simulink subsystem "TV_FLC_V2"  (R2026a)
settings: Solver=VariableStepAuto
model mask{MotorT=Control.MotorTrq, Gr=Control.GearRatio, MotorW=Control.MotorW, rwheel=Control.WheelRad, tr=Control.RearTrack, a=Control.FrontTrackToCG, a_cop=Control.FrontTrackToCoP, Af=Control.FrontalArea, cd=Control.LiftCoef, g=Control.GravitationalAcc, ro=Control.AirDensity, m=Control.Mass, h_CG=Control.CGHeight, L=Control.Wheelbase, Gain=aSteerRatio, Ku=Control.Ku, F=Control.F, P=Control.Proportional_P, I=Control.Integral_I, D=Control.Derivative_D, N=0, Load_Ref=Control.LoadRef, Slip_Ref=Control.SlipRef, FIS_1=Control.FuzzySystem, FIS_2=0, FIS_3=0, vx_th=vx_th, Tmax=max(Control.MotorTrq), C_alpha_F=Control.CalphaF}
  mask prompts: MotorT "Motor Torque:"; Gr "Gear Ratio:"; MotorW "Motor RPM:"; rwheel "Wheel Radius:"; tr "Rear Track:"; a "Front Track to CG:"; a_cop "Front Track to CoP"; Af "Frontal Area:"; cd "Lift Coef:"; g "Graviational ACc"; ro "Air Density:"; m "Mass:"; h_CG "CG Height:"; L "Wheelbase:"; Gain "Simulink:blkprm_prompts:GainGain"; Ku "Understeer Gradient:"; F "Moment to Torque"; P "Simulink:masks:ProportionalP_MP"; I "Simulink:masks:IntegralI_MP"; D "Simulink:masks:DerivativeD_MP"; N "Filter (N):"; Load_Ref "Reference Load Table:"; Slip_Ref "Reference Slip Table:"; FIS_1 "Fuzzy Inference System Var1:"; FIS_2 "Fuzzy Inference System Var2:"; FIS_3 "Fuzzy Inference System Var3:"; vx_th "Activation Velocity:"; Tmax "Max Torque"; C_alpha_F "Front Cornering Stiffness:"
values from neighbouring files (symbols this model uses):
  a = -Vehicle.Chassis.Body.sCG.Value(1)    [sm_car_controlparam_FLCDYC_V2.m]
  Gr = 1/Vehicle.Powertrain.Driveline.Gearbox.ratio.Value    [sm_car_controlparam_FLCDYC_V2.m]
  L = 1.578    [sm_car_controlparam_FLCDYC_V2.m]
  rwheel = 0.263    [sm_car_controlparam_FLCDYC_V2.m]
  tr = Vehicle.Chassis.Body.TrackRear.Value    [sm_car_controlparam_FLCDYC_V2.m]
libraries: simulink x4, fuzblock x3, slpidlib x2, sl_discontinuities x1
settings Model: Creator=andrei  LastModifiedBy=andrei

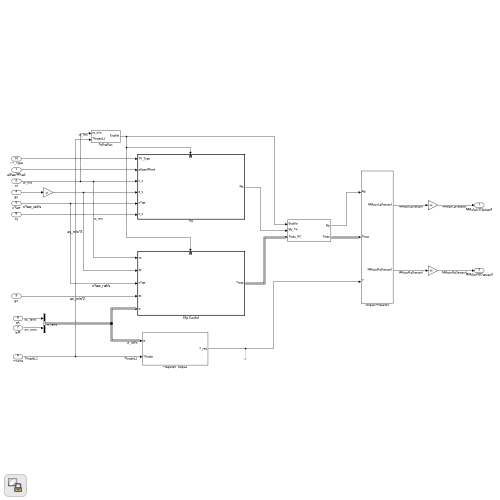
[thumbnail: Simulink's stored preview of the top-level diagram]
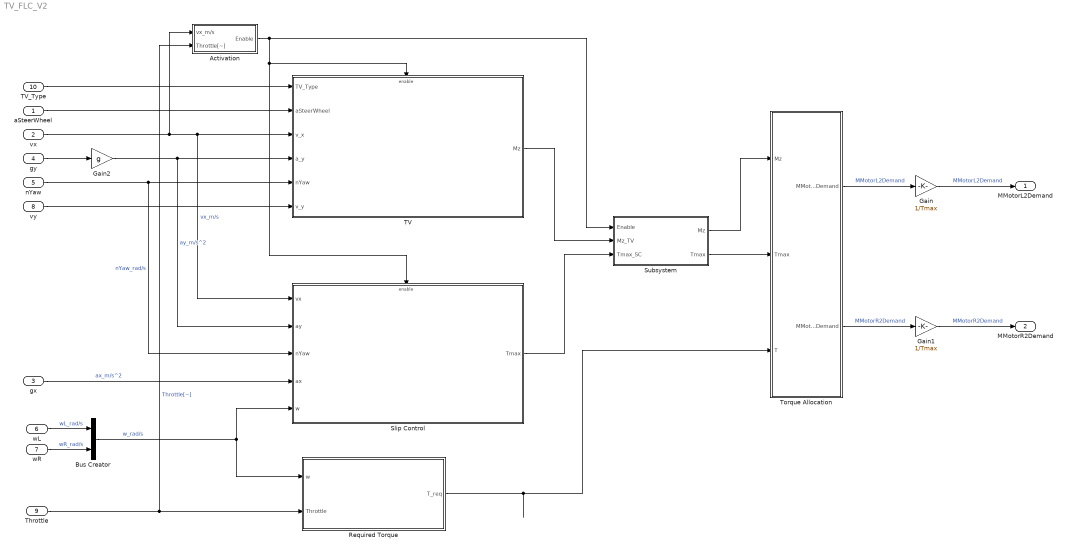
== system TV_FLC_V2 ==
  aSteerWheel : Inport  OutDataTypeStr=double  PortDimensions=1  SampleTime=0
  vx : Inport  Port=2  OutDataTypeStr=double  PortDimensions=1  SampleTime=0
  gx : Inport  Port=3  OutDataTypeStr=double  PortDimensions=1  SampleTime=0
  gy : Inport  Port=4  OutDataTypeStr=double  PortDimensions=1  SampleTime=0
  nYaw : Inport  Port=5  OutDataTypeStr=double  PortDimensions=1  SampleTime=0
  wL : Inport  Port=6  OutDataTypeStr=double  PortDimensions=1  SampleTime=0
  wR : Inport  Port=7  OutDataTypeStr=double  PortDimensions=1  SampleTime=0
  vy : Inport  Port=8  OutDataTypeStr=double  PortDimensions=1  SampleTime=0
  Throttle : Inport  Port=9  OutDataTypeStr=double  PortDimensions=1  SampleTime=0
  TV_Type : Inport  Port=10  OutDataTypeStr=double  PortDimensions=1  SampleTime=0
  Activation : Subsystem
  Bus Creator : BusCreator  Inputs=2
  Gain : Gain  Gain=1/Tmax
  Gain1 : Gain  Gain=1/Tmax
  Gain2 : Gain  Gain=g
  Required Torque : Subsystem
  Slip Control : Subsystem
  Subsystem : Subsystem
  TV : Subsystem
  Torque Allocation : Subsystem
  MMotorL2Demand : Outport  OutDataTypeStr=double  PortDimensions=1  SampleTime=0
  MMotorR2Demand : Outport  Port=2  OutDataTypeStr=double  PortDimensions=1  SampleTime=0
  wires:
  Torque Allocation/1(MMotorL2Demand) -> Gain/1  "MMotorL2Demand"
  wL/1 -> Bus Creator/1  "wL_rad/s"
  gy/1 -> Gain2/1
  Gain1/1 -> MMotorR2Demand/1  "MMotorR2Demand"
  Gain/1 -> MMotorL2Demand/1  "MMotorL2Demand"
  Torque Allocation/2(MMotorR2Demand) -> Gain1/1  "MMotorR2Demand"
  wR/1 -> Bus Creator/2  "wR_rad/s"
  Slip Control/1(Tmax) -> Subsystem/3(Tmax_SC)
  Required Torque/1(T_req) -> Torque Allocation/3(T)
  aSteerWheel/1 -> TV/2(aSteerWheel)
  Gain2/1 -> TV/4(a_y), Slip Control/2(ay)  "ay_m/s^2"
  Bus Creator/1 -> Slip Control/5(w), Required Torque/1(w)  "w_rad/s"
  nYaw/1 -> TV/5(nYaw), Slip Control/3(nYaw)  "nYaw_rad/s"
  gx/1 -> Slip Control/4(ax)  "ax_m/s^2"
  Throttle/1 -> Activation/2(Throttle[~]), Required Torque/2(Throttle)  "Throttle[~]"
  TV/1(Mz) -> Subsystem/2(Mz_TV)
  vy/1 -> TV/6(v_y)
  vx/1 -> TV/3(v_x), Slip Control/1(vx), Activation/1(vx_m/s)  "vx_m/s"
  Activation/1(Enable) -> Slip Control/Enable, TV/Enable, Subsystem/1(Enable)
  Subsystem/1(Mz) -> Torque Allocation/1(Mz)
  Subsystem/2(Tmax) -> Torque Allocation/2(Tmax)
  TV_Type/1 -> TV/1(TV_Type)

== system TV_FLC_V2/Activation ==
  vx_m/s : Inport
  Throttle[~] : Inport  Port=2
  AND : Logic  AllPortsSameDT=off  OutDataTypeStr=boolean
  Compare To Zero : simulink/Logic and Bit Operations/Compare To Zero  relop=~=  OutDataTypeStr=boolean
  Relational Operator : RelationalOperator  Operator=<=  OutDataTypeStr=boolean  RndMeth=Simplest  InputSameDT=off
  th_vx_min : Constant  Value=vx_th
  Enable : Outport
  wires:
  Compare To Zero/1 -> AND/2
  AND/1 -> Enable/1
  Throttle[~]/1 -> Compare To Zero/1
  th_vx_min/1 -> Relational Operator/1
  vx_m/s/1 -> Relational Operator/2
  Relational Operator/1 -> AND/1

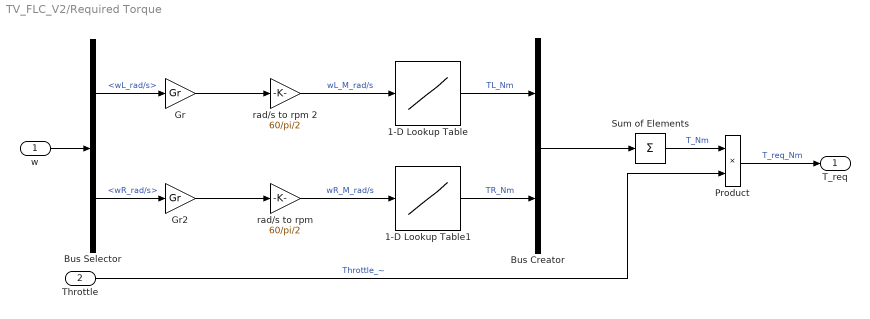
== system TV_FLC_V2/Required Torque ==
  w : Inport
  Throttle : Inport  Port=2
  1-D Lookup Table : Lookup_n-D  NumberOfTableDimensions=1  BreakpointsForDimension1=MotorW  Table=MotorT  InternalRulePriority=Speed  RndMeth=Simplest
  1-D Lookup Table1 : Lookup_n-D  NumberOfTableDimensions=1  BreakpointsForDimension1=MotorW  Table=MotorT  InternalRulePriority=Speed  RndMeth=Simplest
  Bus Creator : BusCreator  Inputs=2
  Bus Selector : BusSelector  OutputSignals=wL_rad/s,wR_rad/s
  Gr : Gain  Gain=Gr
  Gr2 : Gain  Gain=Gr
  Product : Product
  Sum of Elements : Sum  Inputs=+
  rad/s to rpm : Gain  Gain=60/pi/2
  rad/s to rpm 2 : Gain  Gain=60/pi/2
  T_req : Outport
  wires:
  Gr2/1 -> rad/s to rpm/1
  Gr/1 -> rad/s to rpm 2/1
  Bus Creator/1 -> Sum of Elements/1
  1-D Lookup Table/1 -> Bus Creator/1  "TL_Nm"
  rad/s to rpm 2/1 -> 1-D Lookup Table/1  "wL_M_rad/s"
  Bus Selector/2 -> Gr2/1  "<wR_rad/s>"
  Product/1 -> T_req/1  "T_req_Nm"
  Bus Selector/1 -> Gr/1  "<wL_rad/s>"
  rad/s to rpm/1 -> 1-D Lookup Table1/1  "wR_M_rad/s"
  Throttle/1 -> Product/2  "Throttle_~"
  1-D Lookup Table1/1 -> Bus Creator/2  "TR_Nm"
  Sum of Elements/1 -> Product/1  "T_Nm"
  w/1 -> Bus Selector/1

== system TV_FLC_V2/Slip Control ==
  vx : Inport
  ay : Inport  Port=2
  nYaw : Inport  Port=3
  ax : Inport  Port=4
  w : Inport  Port=5
  Enable : EnablePort  StatesWhenEnabling=reset
  Loads : Subsystem
  Maximum Torque Allowed : Subsystem
  Slip Calculation : Subsystem
  Tmax : Outport
  wires:
  w/1 -> Slip Calculation/3(w)  "w_rad/s"
  nYaw/1 -> Slip Calculation/2(nYaw)  "nYaw_rad/s"
  ax/1 -> Loads/1(ax)  "ax_m/s^2"
  Loads/1(Fz) -> Maximum Torque Allowed/1(Fz)
  ay/1 -> Loads/2(ay)  "ay_m/s^2"
  Slip Calculation/2(kappa_rr) -> Maximum Torque Allowed/3(kappa_rr)
  vx/1 -> Loads/3(vx), Slip Calculation/1(Vx)  "vx_m/s"
  Maximum Torque Allowed/1(Tmax) -> Tmax/1
  Slip Calculation/1(kappa_rl) -> Maximum Torque Allowed/2(kappa_rl)

== system TV_FLC_V2/Subsystem ==
  Enable : Inport
  Mz_TV : Inport  Port=2
  Tmax_SC : Inport  Port=3
  Bus Creator1 : BusCreator  Inputs=2
  Constant : Constant  Value=Tmax
  Constant1 : Constant  Value=Tmax
  Constant2 : Constant  Value=0
  Switch : Switch  Criteria=u2 ~= 0  SaturateOnIntegerOverflow=off  InputSameDT=off
  Switch1 : Switch  Criteria=u2 ~= 0  SaturateOnIntegerOverflow=off  InputSameDT=off
  Mz : Outport
  Tmax : Outport  Port=2
  wires:
  Switch1/1 -> Mz/1
  Constant2/1 -> Switch1/3  "Mz"
  Mz_TV/1 -> Switch1/1
  Constant/1 -> Bus Creator1/1  "Tmax_rl_Nm"
  Tmax_SC/1 -> Switch/1
  Bus Creator1/1 -> Switch/3
  Switch/1 -> Tmax/1
  Constant1/1 -> Bus Creator1/2  "Tmax_rr_Nm"
  Enable/1 -> Switch/2, Switch1/2

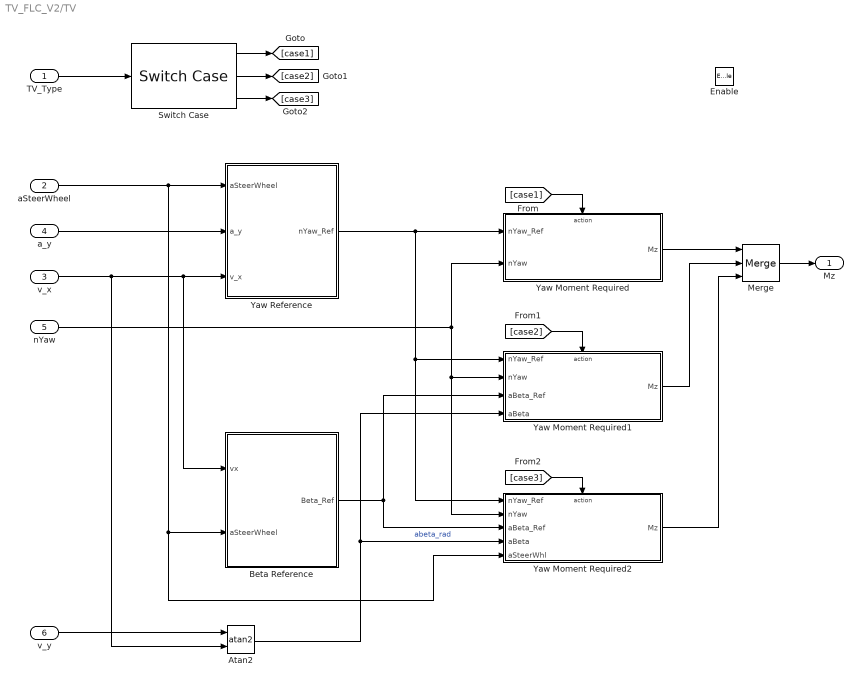
== system TV_FLC_V2/TV ==
  TV_Type : Inport
  aSteerWheel : Inport  Port=2
  v_x : Inport  Port=3
  a_y : Inport  Port=4
  nYaw : Inport  Port=5
  v_y : Inport  Port=6
  Enable : EnablePort  StatesWhenEnabling=reset
  Atan2 : Trigonometry  Operator=atan2
  Beta Reference : Subsystem
  Merge : Merge  Inputs=3
  Switch Case : SwitchCase  CaseConditions={1, 2, 3}  ShowDefaultCase=off
  Yaw Moment Required : Subsystem
  Yaw Moment Required1 : Subsystem
  Yaw Moment Required2 : Subsystem
  Yaw Reference : Subsystem
  Mz : Outport
  wires:
  [case2] -> Yaw Moment Required1/Action
  Merge/1 -> Mz/1
  Yaw Moment Required2/1(Mz) -> Merge/3
  [case3] -> Yaw Moment Required2/Action
  Switch Case/3 -> [case3]
  Switch Case/2 -> [case2]
  [case1] -> Yaw Moment Required/Action
  Switch Case/1 -> [case1]
  Atan2/1 -> Yaw Moment Required2/4(aBeta), Yaw Moment Required1/4(aBeta)  "abeta_rad"
  Yaw Moment Required1/1(Mz) -> Merge/2
  TV_Type/1 -> Switch Case/1
  aSteerWheel/1 -> Yaw Moment Required2/5(aSteerWhl), Beta Reference/2(aSteerWheel), Yaw Reference/1(aSteerWheel)
  v_x/1 -> Yaw Reference/3(v_x), Beta Reference/1(vx), Atan2/2
  nYaw/1 -> Yaw Moment Required1/2(nYaw), Yaw Moment Required2/2(nYaw), Yaw Moment Required/2(nYaw)
  a_y/1 -> Yaw Reference/2(a_y)
  Yaw Moment Required/1(Mz) -> Merge/1
  Yaw Reference/1(nYaw_Ref) -> Yaw Moment Required1/1(nYaw_Ref), Yaw Moment Required2/1(nYaw_Ref), Yaw Moment Required/1(nYaw_Ref)
  Beta Reference/1(Beta_Ref) -> Yaw Moment Required2/3(aBeta_Ref), Yaw Moment Required1/3(aBeta_Ref)
  v_y/1 -> Atan2/1

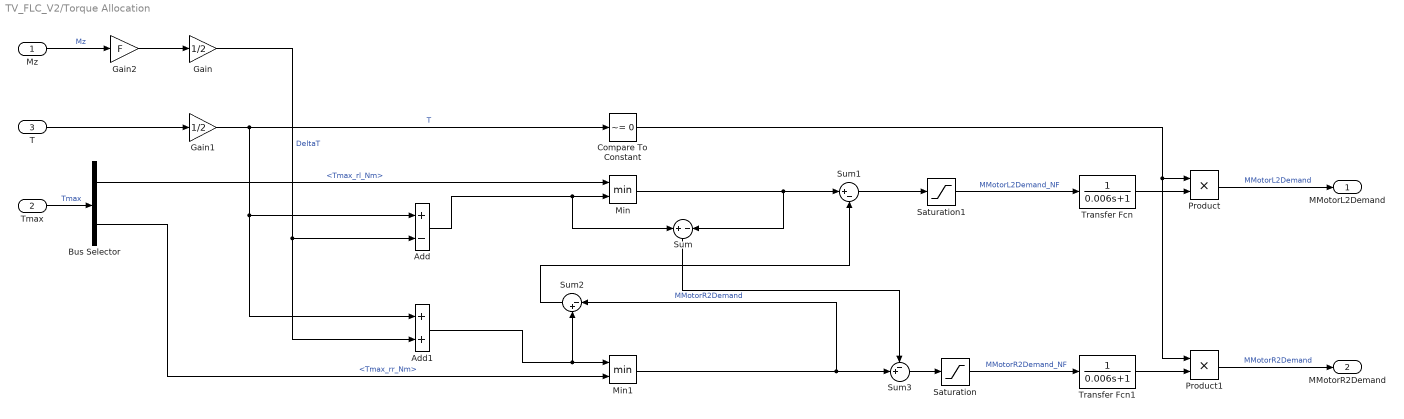
== system TV_FLC_V2/Torque Allocation ==
  Mz : Inport
  Tmax : Inport  Port=2
  T : Inport  Port=3
  Add : Sum  Inputs=+-
  Add1 : Sum
  Bus Selector : BusSelector  OutputSignals=Tmax_rl_Nm,Tmax_rr_Nm
  Compare To Constant : simulink/Logic and Bit Operations/Compare To Constant  relop=~=  const=0  OutDataTypeStr=boolean
  Gain : Gain  Gain=1/2
  Gain1 : Gain  Gain=1/2
  Gain2 : Gain  Gain=F
  Min : MinMax  Inputs=2
  Min1 : MinMax  Inputs=2
  Product : Product
  Product1 : Product
  Saturation : Saturate  UpperLimit=Tmax  LowerLimit=0
  Saturation1 : Saturate  UpperLimit=Tmax  LowerLimit=0
  Sum : Sum  Inputs=+|-
  Sum1 : Sum  Inputs=|+-
  Sum2 : Sum  Inputs=|-+
  Sum3 : Sum  Inputs=-+|
  Transfer Fcn : TransferFcn  Denominator=[0.006 1]
  Transfer Fcn1 : TransferFcn  Denominator=[0.006 1]
  MMotorL2Demand : Outport
  MMotorR2Demand : Outport  Port=2
  wires:
  Saturation1/1 -> Transfer Fcn/1  "MMotorL2Demand_NF"
  Sum3/1 -> Saturation/1
  Sum1/1 -> Saturation1/1
  Gain2/1 -> Gain/1
  Gain/1 -> Add1/2, Add/2  "DeltaT"
  T/1 -> Gain1/1
  Mz/1 -> Gain2/1  "Mz"
  Min/1 -> Sum1/1, Sum/2
  Min1/1 -> Sum2/1, Sum3/2  "MMotorR2Demand"
  Tmax/1 -> Bus Selector/1  "Tmax"
  Bus Selector/1 -> Min/1  "<Tmax_rl_Nm>"
  Bus Selector/2 -> Min1/2  "<Tmax_rr_Nm>"
  Add/1 -> Sum/1, Min/2
  Add1/1 -> Sum2/2, Min1/1
  Sum2/1 -> Sum1/2
  Sum/1 -> Sum3/1
  Gain1/1 -> Compare To Constant/1, Add1/1, Add/1  "T"
  Compare To Constant/1 -> Product/1, Product1/1
  Transfer Fcn/1 -> Product/2
  Product/1 -> MMotorL2Demand/1  "MMotorL2Demand"
  Saturation/1 -> Transfer Fcn1/1  "MMotorR2Demand_NF"
  Transfer Fcn1/1 -> Product1/2
  Product1/1 -> MMotorR2Demand/1  "MMotorR2Demand"

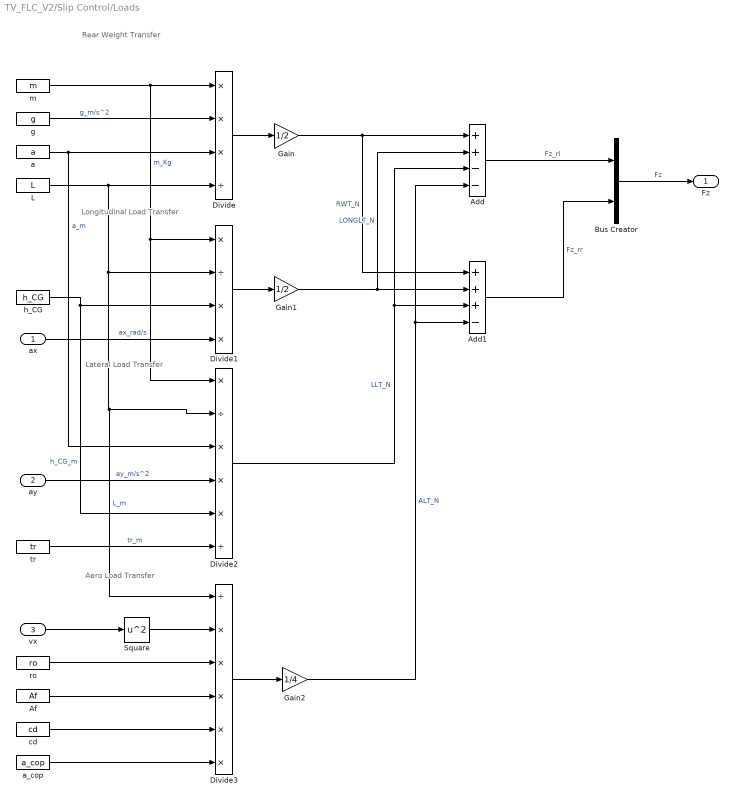
== system TV_FLC_V2/Slip Control/Loads ==
  note: Aero Load Transfer
  note: Lateral Load Transfer
  note: Longitudinal Load Transfer
  note: Rear Weight Transfer
  ax : Inport
  ay : Inport  Port=2
  vx : Inport  Port=3
  Add : Sum  Inputs=++--
  Add1 : Sum  Inputs=+++-
  Af : Constant  Value=Af
  Bus Creator : BusCreator  Inputs=2
  Divide : Product  Inputs=***/
  Divide1 : Product  Inputs=*/**
  Divide2 : Product  Inputs=*/***/
  Divide3 : Product  Inputs=/*****
  Gain : Gain  Gain=1/2
  Gain1 : Gain  Gain=1/2
  Gain2 : Gain  Gain=1/4
  L : Constant  Value=L
  Square : Math  Operator=square
  a : Constant  Value=a
  a_cop : Constant  Value=a_cop
  cd : Constant  Value=cd
  g : Constant  Value=g
  h_CG : Constant  Value=h_CG
  m : Constant  Value=m
  ro : Constant  Value=ro
  tr : Constant  Value=tr
  Fz : Outport
  wires:
  m/1 -> Divide/1, Divide1/1, Divide2/1  "m_Kg"
  g/1 -> Divide/2  "g_m/s^2"
  a/1 -> Divide/3, Divide2/3  "a_m"
  L/1 -> Divide3/1, Divide2/2, Divide1/2, Divide/4  "L_m"
  Divide/1 -> Gain/1
  vx/1 -> Square/1
  Square/1 -> Divide3/2
  Gain/1 -> Add/1, Add1/1  "RWT_N"
  Gain2/1 -> Add/4, Add1/4  "ALT_N"
  h_CG/1 -> Divide2/5, Divide1/3  "h_CG_m"
  ax/1 -> Divide1/4  "ax_rad/s"
  Divide1/1 -> Gain1/1
  Gain1/1 -> Add/2, Add1/2  "LONGLT_N"
  ay/1 -> Divide2/4  "ay_m/s^2"
  tr/1 -> Divide2/6  "tr_m"
  Divide2/1 -> Add/3, Add1/3  "LLT_N"
  Add/1 -> Bus Creator/1  "Fz_rl"
  Add1/1 -> Bus Creator/2  "Fz_rr"
  Bus Creator/1 -> Fz/1  "Fz"
  Divide3/1 -> Gain2/1
  ro/1 -> Divide3/3
  Af/1 -> Divide3/4
  cd/1 -> Divide3/5
  a_cop/1 -> Divide3/6

== system TV_FLC_V2/Slip Control/Maximum Torque Allowed ==
  Fz : Inport
  kappa_rl : Inport  Port=2
  kappa_rr : Inport  Port=3
  Bus Creator : BusCreator  Inputs=2
  Bus Selector : BusSelector  OutputSignals=Fz_rl,Fz_rr
  Slip Correction Left : Subsystem
  Slip Correction Right : Subsystem
  Tmax : Outport
  wires:
  Slip Correction Right/1(Tmax_rr) -> Bus Creator/2  "Tmax_rr_Nm"
  Slip Correction Left/1(Tmax_rl) -> Bus Creator/1  "Tmax_rl_Nm"
  kappa_rl/1 -> Slip Correction Left/1(kappa_rl)
  kappa_rr/1 -> Slip Correction Right/2(kappa_rr)
  Fz/1 -> Bus Selector/1
  Bus Selector/1 -> Slip Correction Left/2(Fz_rl)  "<Fz_rl>"
  Bus Selector/2 -> Slip Correction Right/1(Fz_rr)  "<Fz_rr>"
  Bus Creator/1 -> Tmax/1

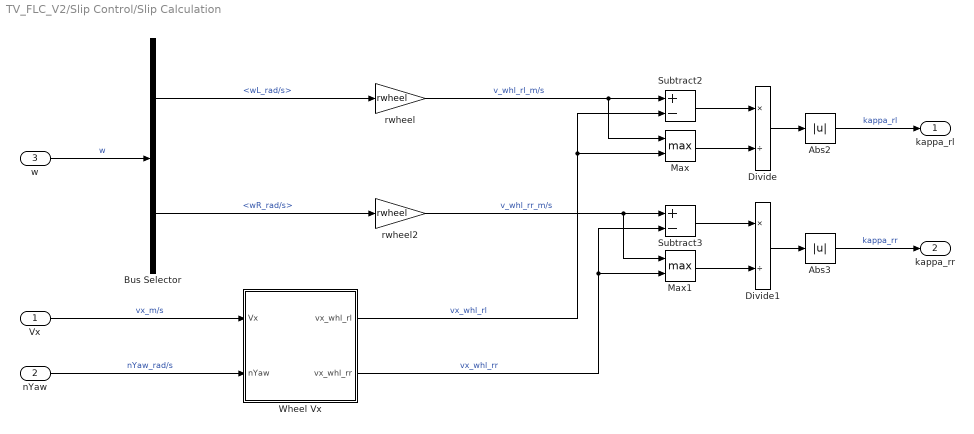
== system TV_FLC_V2/Slip Control/Slip Calculation ==
  Vx : Inport
  nYaw : Inport  Port=2
  w : Inport  Port=3
  Abs2 : Abs  SaturateOnIntegerOverflow=off
  Abs3 : Abs  SaturateOnIntegerOverflow=off
  Bus Selector : BusSelector  OutputSignals=wL_rad/s,wR_rad/s
  Divide : Product  Inputs=*/
  Divide1 : Product  Inputs=*/
  Max : MinMax  Function=max  Inputs=2
  Max1 : MinMax  Function=max  Inputs=2
  Subtract2 : Sum  Inputs=+-
  Subtract3 : Sum  Inputs=+-
  Wheel Vx : Subsystem
  rwheel : Gain  Gain=rwheel
  rwheel2 : Gain  Gain=rwheel
  kappa_rl : Outport
  kappa_rr : Outport  Port=2
  wires:
  Bus Selector/1 -> rwheel/1  "<wL_rad/s>"
  Bus Selector/2 -> rwheel2/1  "<wR_rad/s>"
  Vx/1 -> Wheel Vx/1(Vx)  "vx_m/s"
  w/1 -> Bus Selector/1  "w"
  rwheel/1 -> Max/1, Subtract2/1  "v_whl_rl_m/s"
  rwheel2/1 -> Max1/1, Subtract3/1  "v_whl_rr_m/s"
  nYaw/1 -> Wheel Vx/2(nYaw)  "nYaw_rad/s"
  Abs3/1 -> kappa_rr/1  "kappa_rr"
  Wheel Vx/1(vx_whl_rl) -> Subtract2/2, Max/2  "vx_whl_rl"
  Abs2/1 -> kappa_rl/1  "kappa_rl"
  Subtract2/1 -> Divide/1
  Wheel Vx/2(vx_whl_rr) -> Subtract3/2, Max1/2  "vx_whl_rr"
  Subtract3/1 -> Divide1/1
  Divide/1 -> Abs2/1
  Max/1 -> Divide/2
  Divide1/1 -> Abs3/1
  Max1/1 -> Divide1/2

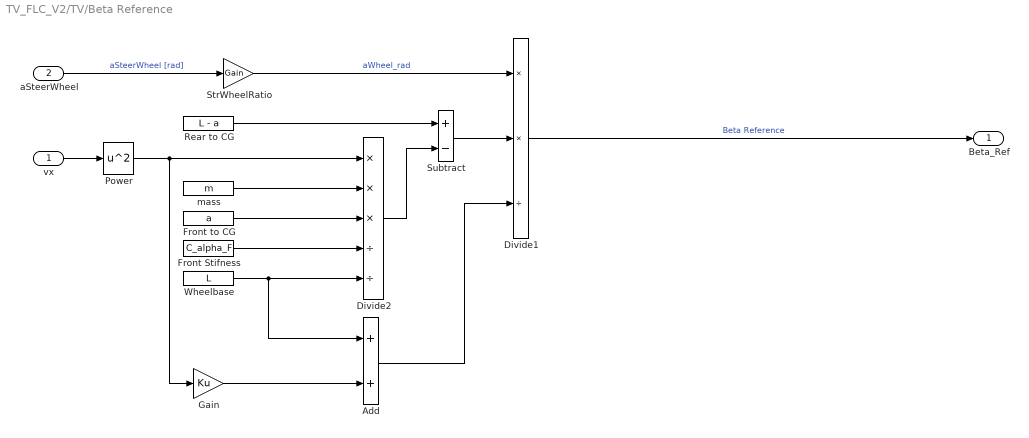
== system TV_FLC_V2/TV/Beta Reference ==
  vx : Inport
  aSteerWheel : Inport  Port=2
  Add : Sum
  Divide1 : Product  Inputs=**/
  Divide2 : Product  Inputs=***//
  Front Stifness : Constant  Value=C_alpha_F
  Front to CG : Constant  Value=a
  Gain : Gain  Gain=Ku
  Power : Math  Operator=square
  Rear to CG : Constant  Value=L - a
  StrWheelRatio : Gain  Gain=Gain
  Subtract : Sum  Inputs=+-
  Wheelbase : Constant  Value=L
  mass : Constant  Value=m
  Beta_Ref : Outport
  wires:
  StrWheelRatio/1 -> Divide1/1  "aWheel_rad"
  Add/1 -> Divide1/3
  Gain/1 -> Add/2
  Power/1 -> Gain/1, Divide2/1
  Divide1/1 -> Beta_Ref/1  "Beta Reference"
  vx/1 -> Power/1
  aSteerWheel/1 -> StrWheelRatio/1  "aSteerWheel [rad]"
  Wheelbase/1 -> Add/1, Divide2/5
  Front Stifness/1 -> Divide2/4
  mass/1 -> Divide2/2
  Front to CG/1 -> Divide2/3
  Rear to CG/1 -> Subtract/1
  Divide2/1 -> Subtract/2
  Subtract/1 -> Divide1/2

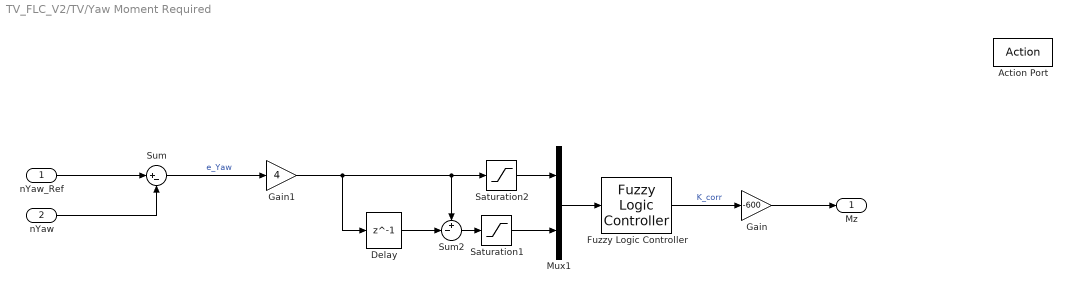
== system TV_FLC_V2/TV/Yaw Moment Required ==
  nYaw_Ref : Inport
  nYaw : Inport  Port=2
  Action Port : ActionPort
  Delay : Delay  DelayLength=1  InputProcessing=Columns as channels (frame based)
  Fuzzy Logic Controller : fuzblock/Fuzzy Logic  Controller  FIS=FIS_1  OutputSampleNumber=101  DataType=double  UseLookupTable=off  NumBreakpoints=10  FuzzifiedInputs=off  RuleFiringStrengths=off  RuleOutputs=off  AggregatedOutputs=off  SimulateUsing=Interpreted execution  OutOfRangeInputValueMessage=warning  NoRuleFiredMessage=warning  EmptyOutputFuzzySetMessage=warning
  Gain : Gain  Gain=-600
  Gain1 : Gain  Gain=4
  Mux1 : Mux  Inputs=2
  Saturation1 : Saturate  UpperLimit=1  LowerLimit=-1  ZeroCross=off
  Saturation2 : Saturate  UpperLimit=1  LowerLimit=-1  ZeroCross=off
  Sum : Sum  Inputs=|+-
  Sum2 : Sum  Inputs=+-|
  Mz : Outport
  wires:
  Gain1/1 -> Delay/1, Saturation2/1, Sum2/1
  Mux1/1 -> Fuzzy Logic Controller/1
  Sum2/1 -> Saturation1/1
  Delay/1 -> Sum2/2
  Saturation2/1 -> Mux1/1
  Saturation1/1 -> Mux1/2
  Gain/1 -> Mz/1
  Fuzzy Logic Controller/1 -> Gain/1  "K_corr"
  nYaw_Ref/1 -> Sum/1
  nYaw/1 -> Sum/2
  Sum/1 -> Gain1/1  "e_Yaw"

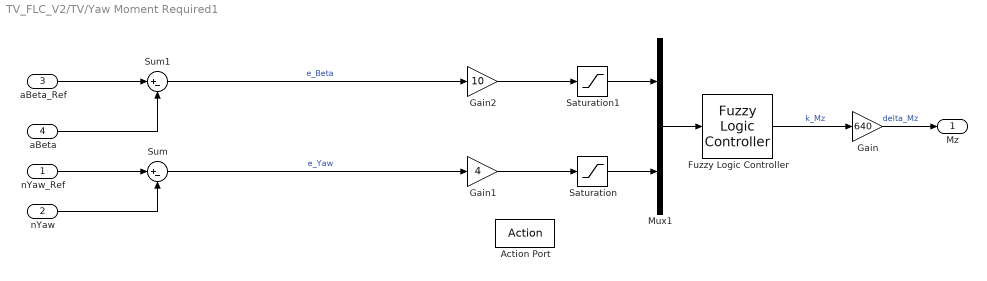
== system TV_FLC_V2/TV/Yaw Moment Required1 ==
  nYaw_Ref : Inport
  nYaw : Inport  Port=2
  aBeta_Ref : Inport  Port=3
  aBeta : Inport  Port=4
  Action Port : ActionPort
  Fuzzy Logic Controller : fuzblock/Fuzzy Logic  Controller  FIS=FIS_2  OutputSampleNumber=101  DataType=double  UseLookupTable=off  NumBreakpoints=10  FuzzifiedInputs=off  RuleFiringStrengths=off  RuleOutputs=off  AggregatedOutputs=off  SimulateUsing=Interpreted execution  OutOfRangeInputValueMessage=warning  NoRuleFiredMessage=warning  EmptyOutputFuzzySetMessage=warning
  Gain : Gain  Gain=640
  Gain1 : Gain  Gain=4
  Gain2 : Gain  Gain=10
  Mux1 : Mux  Inputs=2
  Saturation : Saturate  UpperLimit=1  LowerLimit=-1  ZeroCross=off
  Saturation1 : Saturate  UpperLimit=1  LowerLimit=-1  ZeroCross=off
  Sum : Sum  Inputs=|+-
  Sum1 : Sum  Inputs=|+-
  Mz : Outport
  wires:
  Saturation1/1 -> Mux1/1
  Saturation/1 -> Mux1/2
  Sum1/1 -> Gain2/1  "e_Beta"
  aBeta/1 -> Sum1/2
  aBeta_Ref/1 -> Sum1/1
  Sum/1 -> Gain1/1  "e_Yaw"
  nYaw/1 -> Sum/2
  nYaw_Ref/1 -> Sum/1
  Fuzzy Logic Controller/1 -> Gain/1  "k_Mz"
  Gain/1 -> Mz/1  "delta_Mz"
  Mux1/1 -> Fuzzy Logic Controller/1
  Gain2/1 -> Saturation1/1
  Gain1/1 -> Saturation/1

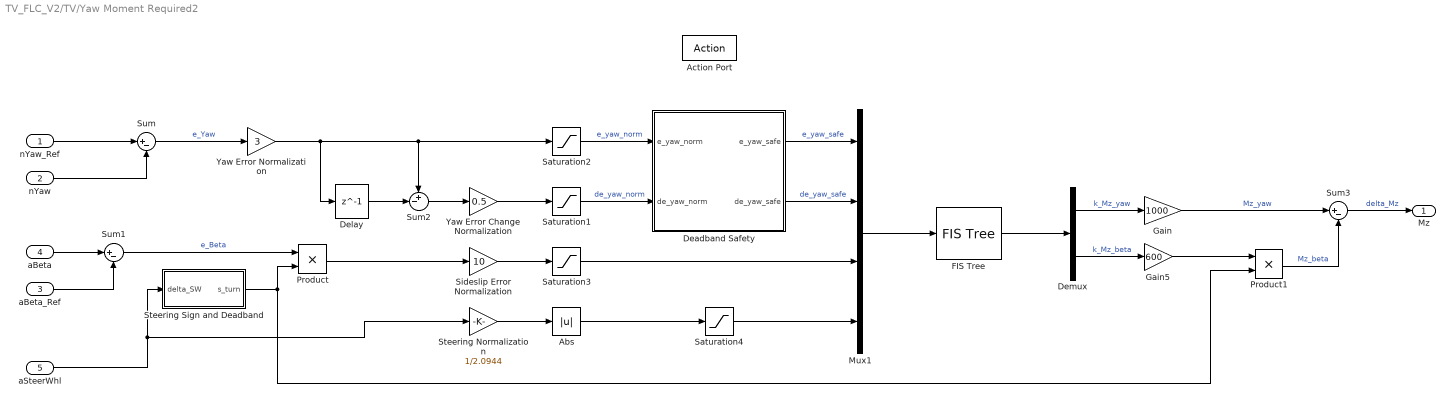
== system TV_FLC_V2/TV/Yaw Moment Required2 ==
  nYaw_Ref : Inport
  nYaw : Inport  Port=2
  aBeta_Ref : Inport  Port=3
  aBeta : Inport  Port=4
  aSteerWhl : Inport  Port=5
  Action Port : ActionPort
  " Yaw Error Change Normalization" : Gain  Gain=0.5
  Abs : Abs  ZeroCross=off  SaturateOnIntegerOverflow=off
  Deadband Safety : Subsystem
  Delay : Delay  DelayLength=1  InputProcessing=Columns as channels (frame based)
  Demux : Demux  Outputs=2
  FIS Tree : fuzblock/FIS Tree  FIS=FIS_3  OutputSampleNumber=101  DataType=single  SimulateUsing=Interpreted execution  OutOfRangeInputValueMessage=warning  NoRuleFiredMessage=warning  EmptyOutputFuzzySetMessage=warning
  Gain : Gain  Gain=1000
  Gain5 : Gain  Gain=600
  Mux1 : Mux
  Product : Product
  Product1 : Product
  Saturation{1..4} (4 alike) : Saturate  UpperLimit=1  LowerLimit=-1  ZeroCross=off
  Sideslip Error Normalization : Gain  Gain=10
  Steering Normalization : Gain  Gain=1/2.0944
  Steering Sign and Deadband : MATLAB Function  TreatAsAtomicUnit=on  mask{delta_th=2}
      mask prompts: delta_th "Steering Th"
  Sum : Sum  Inputs=|+-
  Sum1 : Sum  Inputs=|+-
  Sum2 : Sum  Inputs=+-|
  Sum3 : Sum  Inputs=|+-
  Yaw Error Normalization : Gain  Gain=3
  Mz : Outport
  wires:
  Deadband Safety/2(de_yaw_safe) -> Mux1/2  "de_yaw_safe"
  Deadband Safety/1(e_yaw_safe) -> Mux1/1  "e_yaw_safe"
  Saturation1/1 -> Deadband Safety/2(de_yaw_norm)  "de_yaw_norm"
  Saturation2/1 -> Deadband Safety/1(e_yaw_norm)  "e_yaw_norm"
  Abs/1 -> Saturation4/1
  Product1/1 -> Sum3/2  "Mz_beta"
  Gain5/1 -> Product1/1
  Sum3/1 -> Mz/1  "delta_Mz"
  Demux/2 -> Gain5/1  "k_Mz_beta"
  Demux/1 -> Gain/1  "k_Mz_yaw"
  Product/1 -> Sideslip Error Normalization/1
  Steering Sign and Deadband/1(s_turn) -> Product1/2, Product/2
  " Yaw Error Change Normalization"/1 -> Saturation1/1
  Saturation4/1 -> Mux1/4
  Saturation3/1 -> Mux1/3
  Steering Normalization/1 -> Abs/1
  Sideslip Error Normalization/1 -> Saturation3/1
  Yaw Error Normalization/1 -> Delay/1, Saturation2/1, Sum2/1
  aSteerWhl/1 -> Steering Normalization/1, Steering Sign and Deadband/1(delta_SW)
  aBeta_Ref/1 -> Sum1/2
  aBeta/1 -> Sum1/1
  Sum1/1 -> Product/1  "e_Beta"
  Mux1/1 -> FIS Tree/1
  Sum2/1 -> " Yaw Error Change Normalization"/1
  Delay/1 -> Sum2/2
  Gain/1 -> Sum3/1  "Mz_yaw"
  FIS Tree/1 -> Demux/1
  nYaw_Ref/1 -> Sum/1
  nYaw/1 -> Sum/2
  Sum/1 -> Yaw Error Normalization/1  "e_Yaw"

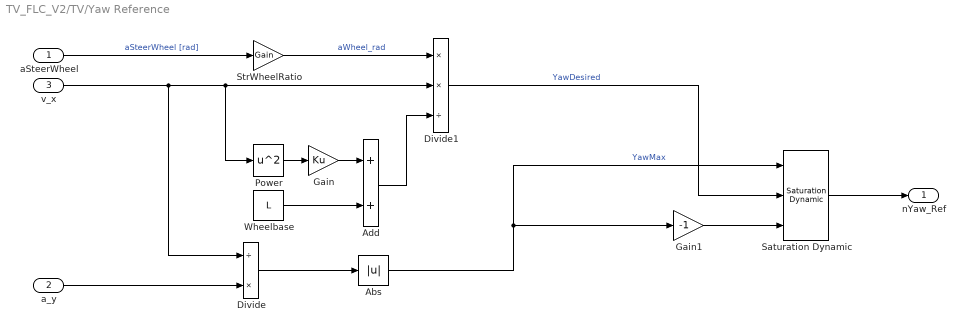
== system TV_FLC_V2/TV/Yaw Reference ==
  aSteerWheel : Inport
  a_y : Inport  Port=2
  v_x : Inport  Port=3
  Abs : Abs  SaturateOnIntegerOverflow=off
  Add : Sum
  Divide : Product  Inputs=/*
  Divide1 : Product  Inputs=**/
  Gain : Gain  Gain=Ku
  Gain1 : Gain  Gain=-1
  Power : Math  Operator=square
  Saturation Dynamic : sl_discontinuities/Saturation Dynamic  OutMin=[]  OutMax=[]  OutDataTypeStr=Inherit: Same as second input  OutDataType=fixdt(1, 16)  OutScaling=2^-10  DoSatur=off
  StrWheelRatio : Gain  Gain=Gain
  Wheelbase : Constant  Value=L
  nYaw_Ref : Outport
  wires:
  StrWheelRatio/1 -> Divide1/1  "aWheel_rad"
  aSteerWheel/1 -> StrWheelRatio/1  "aSteerWheel [rad]"
  v_x/1 -> Divide1/2, Power/1, Divide/1
  a_y/1 -> Divide/2
  Divide/1 -> Abs/1
  Saturation Dynamic/1 -> nYaw_Ref/1
  Abs/1 -> Saturation Dynamic/1, Gain1/1  "YawMax"
  Gain1/1 -> Saturation Dynamic/3
  Divide1/1 -> Saturation Dynamic/2  "YawDesired"
  Power/1 -> Gain/1
  Gain/1 -> Add/1
  Wheelbase/1 -> Add/2
  Add/1 -> Divide1/3

== system TV_FLC_V2/Slip Control/Maximum Torque Allowed/Slip Correction Left ==
  kappa_rl : Inport
  Fz_rl : Inport  Port=2
  1-D Lookup Table : Lookup_n-D  NumberOfTableDimensions=1  BreakpointsForDimension1=Load_Ref  Table=Slip_Ref  ExtrapMethod=Clip  UseLastTableValue=on  InternalRulePriority=Speed  RndMeth=Simplest
  PID Controller : slpidlib/PID Controller  Controller=PID  Form=Parallel  TimeDomain=Discrete-time  UseExternalTs=off  SampleTime=0.005  IntegratorMethod=Forward Euler  FilterMethod=Forward Euler  ControllerParametersSource=internal  P=P  I=I  UseKiTs=off  D=D  UseExternalDerivativeSource=off  N=30  UseFilter=on  TunerSelectOption=Transfer Function Based (PID Tuner App)  InitialConditionSource=internal  InitialConditionForIntegrator=Tmax  InitialConditionForFilter=0  DifferentiatorICPrevScaledInput=Tmax  ExternalReset=none  TrackingMode=off  Kt=1  LimitOutput=on  SatLimitsSource=internal  UpperSaturationLimit=Tmax  LowerSaturationLimit=0  LinearizeAsGain=on  AntiWindupMode=clamping  Kb=1  LimitIntegrator=off  UpperIntegratorSaturationLimit=inf  LowerIntegratorSaturationLimit=-inf  POutMin=[]  POutMax=[]  IOutMin=[]  IOutMax=[]  DOutMin=[]  DOutMax=[]  NOutMin=[]  NOutMax=[]  SumOutMin=[]  SumOutMax=[]  SaturationOutMin=[]  SaturationOutMax=[]  PParamMin=[]  PParamMax=[]  IParamMin=[]  IParamMax=[]  DParamMin=[]  DParamMax=[]  NParamMin=[]  NParamMax=[]  KbParamMin=[]  KbParamMax=[]  KtParamMin=[]  KtParamMax=[]  KbOutMin=[]  KbOutMax=[]  KtOutMin=[]  KtOutMax=[]  IntegratorOutMin=[]  IntegratorOutMax=[]  FilterOutMin=[]  FilterOutMax=[]  SumI1OutMin=[]  SumI1OutMax=[]  SumI2OutMin=[]  SumI2OutMax=[]  SumI3OutMin=[]  SumI3OutMax=[]  SumI4OutMin=[]  SumI4OutMax=[]  SumDOutMin=[]  SumDOutMax=[]  DifferentiatorOutMin=[]  DifferentiatorOutMax=[]  FilterDiffOutCoefMin=[]  FilterDiffOutCoefMax=[]  ReciprocalOutMin=[]  ReciprocalOutMax=[]  SumDenOutMin=[]  SumDenOutMax=[]  SumNumOutMin=[]  SumNumOutMax=[]  DivideOutMin=[]  DivideOutMax=[]  UdiffTsProdOutMin=[]  UdiffTsProdOutMax=[]  NTsProdOutMin=[]  NTsProdOutMax=[]  UintegralTsProdOutMin=[]  UintegralTsProdOutMax=[]  UngainTsProdOutMin=[]  UngainTsProdOutMax=[]  ClampingZeroOutDataTypeStr=Inherit: Inherit via back propagation  ClampingZeroOutMin=[]  ClampingZeroOutMax=[]  FilterDenConstantOutDataTypeStr=Inherit: Inherit via back propagation  FilterDenConstantOutMin=[]  FilterDenConstantOutMax=[]  PCopyOutDataTypeStr=Inherit: Inherit via back propagation  PCopyOutMin=[]  PCopyOutMax=[]  NCopyOutDataTypeStr=Inherit: Inherit via back propagation  NCopyOutMin=[]  NCopyOutMax=[]  IntegratorContinuousStateAttributes=''  IntegratorStateMustResolveToSignalObject=off  IntegratorRTWStateStorageClass=Auto  FilterContinuousStateAttributes=''  FilterStateMustResolveToSignalObject=off  FilterRTWStateStorageClass=Auto  ParallelPVariant=InternalParameters  IdealPVariant=Disabled  IVariant=InternalParameters  DVariant=InternalParameters  IntegratorVariant=Discrete  SatVariant=Enabled  AWVariant=DiscClampingParallel  PCopyVariant=Disabled  TRVariant=Disabled  FdbkBlocksVariant=Forward  IdealPFdbkVariant=Disabled  SatFdbkVariant=Disabled  DerivativeFilterVariant=ForwardEulerFilter  NVariant=InternalParameters  NCopyVariant=Disabled  FilterICVariant=InternalICsFilter  IntegratorICVariant=InternalICs  ExternalResetVariant=Disabled  TRSumVariant=Passthrough  SumFdbkVariant=Disabled  SumVariant=Sum_PID  TsampFilterVariant=InternalTs  TsampNgainVariant=Passthrough  TsampIntegralVariant=Disabled_SignalSpec  ExternalSaturationOutDataTypeStr=Inherit: Same as second input  DerivativeSourceVariant=ErrorSignal  PreIntVariant=InternalPreInt
  Sum : Sum  Inputs=|+-
  Tmax_rl : Outport
  wires:
  PID Controller/1 -> Tmax_rl/1  "Tmax_rl_Nm"
  kappa_rl/1 -> Sum/2  "kappa_rl"
  1-D Lookup Table/1 -> Sum/1  "kappa_ref"
  Sum/1 -> PID Controller/1  "e"
  Fz_rl/1 -> 1-D Lookup Table/1  "Fz_rl_N"

== system TV_FLC_V2/Slip Control/Maximum Torque Allowed/Slip Correction Right ==
  Fz_rr : Inport
  kappa_rr : Inport  Port=2
  1-D Lookup Table : Lookup_n-D  NumberOfTableDimensions=1  BreakpointsForDimension1=Load_Ref  Table=Slip_Ref  ExtrapMethod=Clip  UseLastTableValue=on  InternalRulePriority=Speed  RndMeth=Simplest
  PID Controller : slpidlib/PID Controller  Controller=PID  Form=Parallel  TimeDomain=Discrete-time  UseExternalTs=off  SampleTime=0.005  IntegratorMethod=Forward Euler  FilterMethod=Forward Euler  ControllerParametersSource=internal  P=P  I=I  UseKiTs=off  D=D  UseExternalDerivativeSource=off  N=30  UseFilter=on  TunerSelectOption=Transfer Function Based (PID Tuner App)  InitialConditionSource=internal  InitialConditionForIntegrator=Tmax  InitialConditionForFilter=0  DifferentiatorICPrevScaledInput=Tmax  ExternalReset=none  TrackingMode=off  Kt=1  LimitOutput=on  SatLimitsSource=internal  UpperSaturationLimit=Tmax  LowerSaturationLimit=0  LinearizeAsGain=on  AntiWindupMode=clamping  Kb=1  LimitIntegrator=off  UpperIntegratorSaturationLimit=inf  LowerIntegratorSaturationLimit=-inf  POutMin=[]  POutMax=[]  IOutMin=[]  IOutMax=[]  DOutMin=[]  DOutMax=[]  NOutMin=[]  NOutMax=[]  SumOutMin=[]  SumOutMax=[]  SaturationOutMin=[]  SaturationOutMax=[]  PParamMin=[]  PParamMax=[]  IParamMin=[]  IParamMax=[]  DParamMin=[]  DParamMax=[]  NParamMin=[]  NParamMax=[]  KbParamMin=[]  KbParamMax=[]  KtParamMin=[]  KtParamMax=[]  KbOutMin=[]  KbOutMax=[]  KtOutMin=[]  KtOutMax=[]  IntegratorOutMin=[]  IntegratorOutMax=[]  FilterOutMin=[]  FilterOutMax=[]  SumI1OutMin=[]  SumI1OutMax=[]  SumI2OutMin=[]  SumI2OutMax=[]  SumI3OutMin=[]  SumI3OutMax=[]  SumI4OutMin=[]  SumI4OutMax=[]  SumDOutMin=[]  SumDOutMax=[]  DifferentiatorOutMin=[]  DifferentiatorOutMax=[]  FilterDiffOutCoefMin=[]  FilterDiffOutCoefMax=[]  ReciprocalOutMin=[]  ReciprocalOutMax=[]  SumDenOutMin=[]  SumDenOutMax=[]  SumNumOutMin=[]  SumNumOutMax=[]  DivideOutMin=[]  DivideOutMax=[]  UdiffTsProdOutMin=[]  UdiffTsProdOutMax=[]  NTsProdOutMin=[]  NTsProdOutMax=[]  UintegralTsProdOutMin=[]  UintegralTsProdOutMax=[]  UngainTsProdOutMin=[]  UngainTsProdOutMax=[]  ClampingZeroOutDataTypeStr=Inherit: Inherit via back propagation  ClampingZeroOutMin=[]  ClampingZeroOutMax=[]  FilterDenConstantOutDataTypeStr=Inherit: Inherit via back propagation  FilterDenConstantOutMin=[]  FilterDenConstantOutMax=[]  PCopyOutDataTypeStr=Inherit: Inherit via back propagation  PCopyOutMin=[]  PCopyOutMax=[]  NCopyOutDataTypeStr=Inherit: Inherit via back propagation  NCopyOutMin=[]  NCopyOutMax=[]  IntegratorContinuousStateAttributes=''  IntegratorStateMustResolveToSignalObject=off  IntegratorRTWStateStorageClass=Auto  FilterContinuousStateAttributes=''  FilterStateMustResolveToSignalObject=off  FilterRTWStateStorageClass=Auto  ParallelPVariant=InternalParameters  IdealPVariant=Disabled  IVariant=InternalParameters  DVariant=InternalParameters  IntegratorVariant=Discrete  SatVariant=Enabled  AWVariant=DiscClampingParallel  PCopyVariant=Disabled  TRVariant=Disabled  FdbkBlocksVariant=Forward  IdealPFdbkVariant=Disabled  SatFdbkVariant=Disabled  DerivativeFilterVariant=ForwardEulerFilter  NVariant=InternalParameters  NCopyVariant=Disabled  FilterICVariant=InternalICsFilter  IntegratorICVariant=InternalICs  ExternalResetVariant=Disabled  TRSumVariant=Passthrough  SumFdbkVariant=Disabled  SumVariant=Sum_PID  TsampFilterVariant=InternalTs  TsampNgainVariant=Passthrough  TsampIntegralVariant=Disabled_SignalSpec  ExternalSaturationOutDataTypeStr=Inherit: Same as second input  DerivativeSourceVariant=ErrorSignal  PreIntVariant=InternalPreInt
  Sum : Sum  Inputs=|+-
  Tmax_rr : Outport
  wires:
  PID Controller/1 -> Tmax_rr/1  "Tmax_rl_Nm"
  Fz_rr/1 -> 1-D Lookup Table/1  "Fz_rr_N"
  1-D Lookup Table/1 -> Sum/1  "kappa_ref"
  kappa_rr/1 -> Sum/2  "kappa_rr"
  Sum/1 -> PID Controller/1  "e"

== system TV_FLC_V2/Slip Control/Slip Calculation/Wheel Vx ==
  Vx : Inport
  nYaw : Inport  Port=2
  Add : Sum  Inputs=+-
  Add2 : Sum
  Divide : Product  Inputs=**
  Gain : Gain  Gain=1/2
  Rear Track : Constant  Value=tr
  vx_whl_rl : Outport
  vx_whl_rr : Outport  Port=2
  wires:
  Rear Track/1 -> Gain/1  "tr_m"
  nYaw/1 -> Divide/1  "nYaw_rad/s"
  Gain/1 -> Divide/2
  Vx/1 -> Add2/1, Add/1  "vx_m/s"
  Divide/1 -> Add2/2, Add/2
  Add/1 -> vx_whl_rl/1  "vx_whl_rl"
  Add2/1 -> vx_whl_rr/1  "vx_whl_rr"

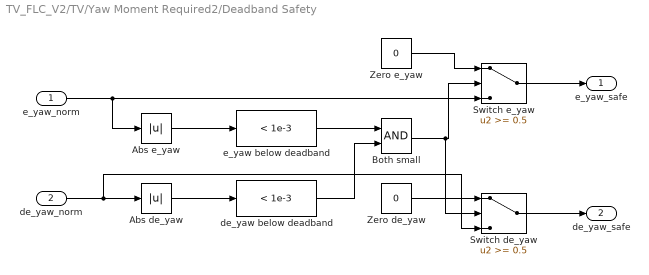
== system TV_FLC_V2/TV/Yaw Moment Required2/Deadband Safety ==
  e_yaw_norm : Inport
  de_yaw_norm : Inport  Port=2
  Abs de_yaw : Abs
  Abs e_yaw : Abs
  Both small : Logic  AllPortsSameDT=off  OutDataTypeStr=boolean
  Switch de_yaw : Switch  Threshold=0.5  ZeroCross=off
  Switch e_yaw : Switch  Threshold=0.5  ZeroCross=off
  Zero de_yaw : Constant  Value=0
  Zero e_yaw : Constant  Value=0
  de_yaw below deadband : simulink/Logic and Bit Operations/Compare To Constant  relop=<  const=1e-3  OutDataTypeStr=boolean  ZeroCross=off
  e_yaw below deadband : simulink/Logic and Bit Operations/Compare To Constant  relop=<  const=1e-3  OutDataTypeStr=boolean  ZeroCross=off
  e_yaw_safe : Outport
  de_yaw_safe : Outport  Port=2
  wires:
  e_yaw_norm/1 -> Switch e_yaw/3, Abs e_yaw/1
  de_yaw_norm/1 -> Switch de_yaw/3, Abs de_yaw/1
  Switch de_yaw/1 -> de_yaw_safe/1
  Abs de_yaw/1 -> de_yaw below deadband/1
  Switch e_yaw/1 -> e_yaw_safe/1
  Abs e_yaw/1 -> e_yaw below deadband/1
  e_yaw below deadband/1 -> Both small/1
  de_yaw below deadband/1 -> Both small/2
  Zero de_yaw/1 -> Switch de_yaw/1
  Zero e_yaw/1 -> Switch e_yaw/1
  Both small/1 -> Switch e_yaw/2, Switch de_yaw/2

== matlab function TV_FLC_V2/TV/Yaw Moment Required2/Steering Sign and Deadband ==
  data: delta_SW input; s_turn output; delta_th parameter
function s_turn = fcn(delta_SW, delta_th)
delta_th = deg2rad(delta_th);
if delta_SW >= delta_th
    s_turn = +1;
elseif delta_SW <= -delta_th
    s_turn = -1;
elseif abs(delta_SW) < delta_th
    s_turn = 0;
else
    s_turn = 0;
end
